simulink model "EXTENSION1"  (R2025b)
settings: Solver=FixedStepAuto  StartTime=0.0  StopTime=10.0  FixedStep=0.001  RelTol=1e-3
undefined symbols (not defined in the file): b, C, c, g, I, kb, KK, kt, l, M, m, r, Rm, sysKF
libraries: simulink x5, vrlib x3
settings Model: Creator=jitendra  LastModifiedBy=joelalfaro
settings DataIOCC: ExternalInput=getinputstruct(op_trim1)  InitialState=getstatestruct(op_trim1)  ReturnWorkspaceOutputs=off
settings DebuggingCC: UnconnectedInputMsg=warning  UnconnectedOutputMsg=warning  UnconnectedLineMsg=warning  ArithmeticOperatorsInVariantConditions=warning
settings ModelReferenceCC: EnableRefExpFcnMdlSchedulingChecks=on
settings SFSimCC: SimUseLocalCustomCode=off  CustomCodeUndefinedFunction=UseInterfaceOnly
settings RTWCC: RTWUseLocalCustomCode=off  GPUComputeCapability=3.5

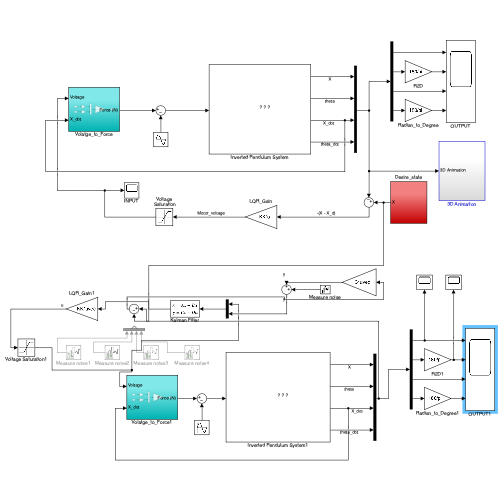
[thumbnail: Simulink's stored preview of the top-level diagram]
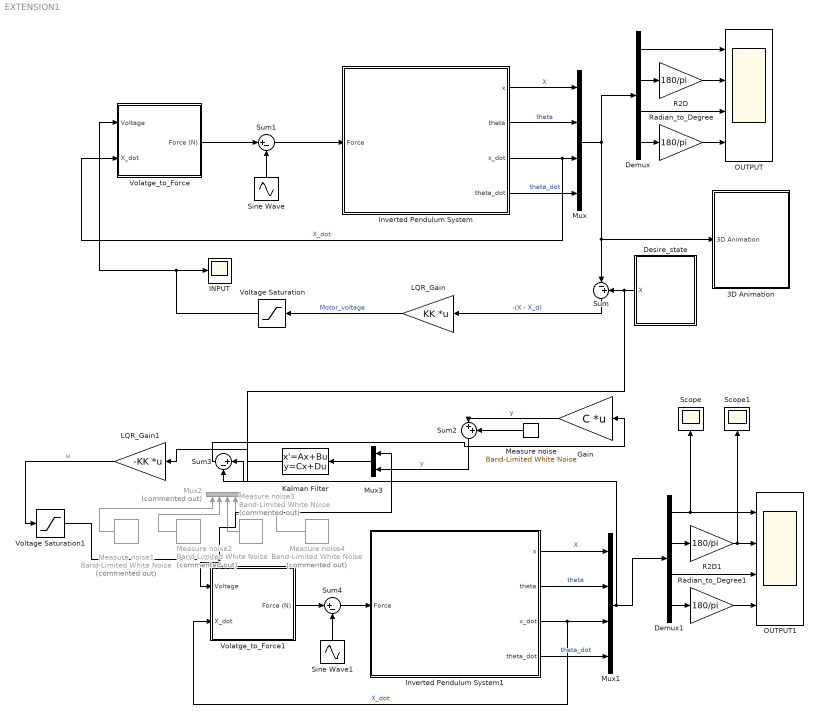
== system EXTENSION1 ==
  3D Animation : Subsystem
  Demux : Demux
  Demux1 : Demux
  Desire_state : Subsystem
  Gain : Gain  Gain=C  Multiplication=Matrix(K*u) (u vector)
  INPUT : Scope
      settings: ActiveDisplayYMinimum=-15  ActiveDisplayYMaximum=15
  Inverted Pendulum System : Subsystem
      mask Display: image('ip_model.png');
  Inverted Pendulum System1 : Subsystem
      mask Display: image('ip_model.png');
  Kalman Filter : StateSpace  A=sysKF.A  B=sysKF.B  C=sysKF.C  D=sysKF.D  InitialCondition=[0.1; 160*(pi/180)-pi; 0; 0]
  LQR_Gain : Gain  Gain=KK  Multiplication=Matrix(K*u)
  LQR_Gain1 : Gain  Gain=-KK  Multiplication=Matrix(K*u) (u vector)
  Measure noise : simulink/Sources/Band-Limited White Noise  Cov=[0]  Ts=1  seed=[23341]
  Measure noise{1..4} (4 alike) : simulink/Sources/Band-Limited White Noise  Commented=on  Cov=[0.05]  Ts=1  seed=[23341]
  Mux : Mux
  Mux1 : Mux
  Mux2 : Mux  Commented=on
  Mux3 : Mux  Inputs=2
  OUTPUT : Scope  NumInputPorts=4
      settings: ActiveDisplayString=4  ActiveDisplayYMinimum=-697.02054851210175  ActiveDisplayYMaximum=832.81658993210158  YLabel=\theta dot (deg/sec)
  OUTPUT1 : Scope  NumInputPorts=4
      settings: ActiveDisplayString=4  ActiveDisplayYMinimum=-175.01239944867373  ActiveDisplayYMaximum=256.9962748777549  YLabel=\theta dot (deg/sec)  DataLoggingVariableName=ScopeData2
  R2D : Gain  Gain=180/pi
  R2D1 : Gain  Gain=180/pi
  Radian_to_Degree : Gain  Gain=180/pi
  Radian_to_Degree1 : Gain  Gain=180/pi
  Scope : Scope
      settings: ActiveDisplayYMinimum=0.030577971463402534  ActiveDisplayYMaximum=0.77691598442287257  DataLoggingVariableName=ScopeData3
  Scope1 : Scope
      settings: ActiveDisplayYMinimum=151.06879515780136  ActiveDisplayYMaximum=200.28914360114618  DataLoggingVariableName=ScopeData4
  Sine Wave : Sin  Amplitude=0  SampleTime=0
  Sine Wave1 : Sin  Amplitude=0  SampleTime=0
  Sum : Sum  Inputs=|-+
  Sum1 : Sum  Inputs=|+-
  Sum2 : Sum  Inputs=|++
  Sum3 : Sum  Inputs=|+-
  Sum4 : Sum  Inputs=|+-
  Volatge_to_Force : Subsystem
  Volatge_to_Force1 : Subsystem
  Voltage Saturation : Saturate  UpperLimit=12  LowerLimit=-12
  Voltage Saturation1 : Saturate  UpperLimit=12  LowerLimit=-12
  wires:
  Inverted Pendulum System/3(x_dot) -> Volatge_to_Force/2(X_dot), Mux/3  "X_dot"
  Inverted Pendulum System/2(theta) -> Mux/2  "theta"
  Inverted Pendulum System/1(x) -> Mux/1  "X"
  Inverted Pendulum System/4(theta_dot) -> Mux/4  "theta_dot"
  Mux/1 -> Demux/1, Sum/1, 3D Animation/1(3D Animation)
  LQR_Gain/1 -> Voltage Saturation/1  "Motor_voltage"
  Desire_state/1(X) -> Sum/2, Sum3/2
  Sum/1 -> LQR_Gain/1  "-(X - X_d)"
  Voltage Saturation/1 -> INPUT/1, Volatge_to_Force/1(Voltage)
  Demux/2 -> R2D/1
  Demux/1 -> OUTPUT/1
  Demux/3 -> OUTPUT/3
  Demux/4 -> Radian_to_Degree/1
  R2D/1 -> OUTPUT/2
  Radian_to_Degree/1 -> OUTPUT/4
  Volatge_to_Force/1(Force (N)) -> Sum1/1
  Sum1/1 -> Inverted Pendulum System/1(Force)
  Sine Wave/1 -> Sum1/2
  Measure noise4/1 -> Mux2/4
  Radian_to_Degree1/1 -> OUTPUT1/4
  Demux1/3 -> OUTPUT1/3
  Measure noise3/1 -> Mux2/3
  Inverted Pendulum System1/1(x) -> Mux1/1  "X"
  Demux1/1 -> OUTPUT1/1, Scope/1
  Sum2/1 -> Mux3/2  "y"
  Inverted Pendulum System1/2(theta) -> Mux1/2  "theta"
  Demux1/4 -> Radian_to_Degree1/1
  Mux3/1 -> Kalman Filter/1
  Mux1/1 -> Demux1/1, Sum3/1
  Gain/1 -> Sum2/1  "y"
  Measure noise2/1 -> Mux2/2
  Inverted Pendulum System1/4(theta_dot) -> Mux1/4  "theta_dot"
  Measure noise1/1 -> Mux2/1
  R2D1/1 -> OUTPUT1/2, Scope1/1
  Demux1/2 -> R2D1/1
  Measure noise/1 -> Sum2/2
  Inverted Pendulum System1/3(x_dot) -> Volatge_to_Force1/2(X_dot), Mux1/3  "X_dot"
  Sine Wave1/1 -> Sum4/2
  Volatge_to_Force1/1(Force (N)) -> Sum4/1
  Sum4/1 -> Inverted Pendulum System1/1(Force)
  Sum3/1 -> Gain/1
  Kalman Filter/1 -> LQR_Gain1/1
  LQR_Gain1/1 -> Voltage Saturation1/1  "u"
  Voltage Saturation1/1 -> Mux3/1, Volatge_to_Force1/1(Voltage)

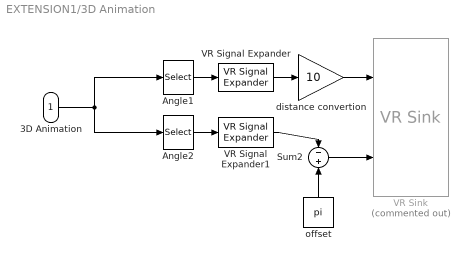
== system EXTENSION1/3D Animation ==
  3D Animation : Inport
  Angle1 : Selector  InputPortWidth=4  IndexOptions=Index vector (dialog)  Indices=[1]  OutputSizes=1
  Angle2 : Selector  InputPortWidth=4  IndexOptions=Index vector (dialog)  Indices=[2]  OutputSizes=1
  Sum2 : Sum  Inputs=-|+
  VR Signal Expander : vrlib/VR Signal Expander  outwidth=3  outidx=[1]
  VR Signal Expander1 : vrlib/VR Signal Expander  outwidth=4  outidx=[4]
  VR Sink : vrlib/VR Sink  Commented=on  InstantiateOnLoad=on  SampleTime=0.02  ViewEnable=on  RemoteChange=off  RemoteView=off  FieldsWritten=cart.translation.3.1.1.double#joint.rotation.4.1.1.double  WorldFileName=Inverted_pendulum12.wrl  AutoView=off  VideoDimensions=[]  AllowVariableSize=off  FigureProperties=[]
  distance convertion : Gain  Gain=10
  offset : Constant  Value=pi
  wires:
  VR Signal Expander/1 -> distance convertion/1
  3D Animation/1 -> Angle2/1, Angle1/1
  Angle1/1 -> VR Signal Expander/1
  Angle2/1 -> VR Signal Expander1/1
  offset/1 -> Sum2/2
  Sum2/1 -> VR Sink/2
  VR Signal Expander1/1 -> Sum2/1
  distance convertion/1 -> VR Sink/1

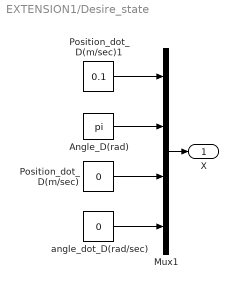
== system EXTENSION1/Desire_state ==
  Angle_D(rad) : Constant  Value=pi
  Mux1 : Mux
  Position_dot_D(m/sec) : Constant  Value=0
  Position_dot_D(m/sec)1 : Constant  Value=0.1
  angle_dot_D(rad/sec) : Constant  Value=0
  X : Outport  VectorParamsAs1DForOutWhenUnconnected=off
  wires:
  Mux1/1 -> X/1
  Position_dot_D(m/sec)/1 -> Mux1/3
  angle_dot_D(rad/sec)/1 -> Mux1/4
  Angle_D(rad)/1 -> Mux1/2
  Position_dot_D(m/sec)1/1 -> Mux1/1

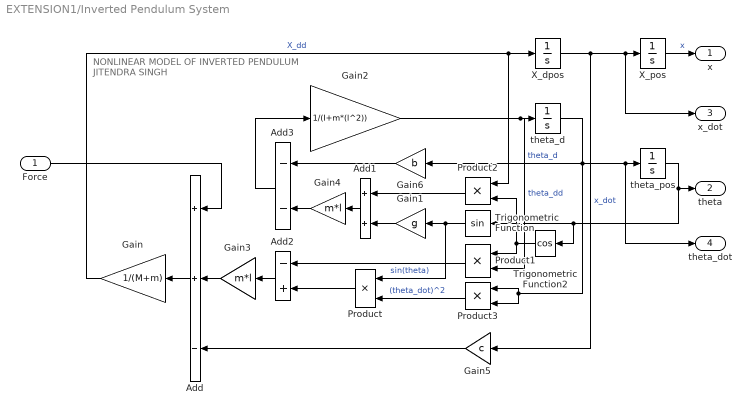
== system EXTENSION1/Inverted Pendulum System ==
  note: NONLINEAR MODEL OF
      | INVERTED PENDULUM
      | JITENDRA SINGH
  Force : Inport
  Add : Sum  Inputs=++-
  Add1 : Sum
  Add2 : Sum  Inputs=-+
  Add3 : Sum  Inputs=--
  Gain : Gain  Gain=1/(M+m)
  Gain1 : Gain  Gain=g
  Gain2 : Gain  Gain=1/(I+m*(l^2))
  Gain3 : Gain  Gain=m*l
  Gain4 : Gain  Gain=m*l
  Gain5 : Gain  Gain=c
  Gain6 : Gain  Gain=b
  Product{,1..3} (4 alike) : Product
  Trigonometric Function : Trigonometry
  Trigonometric Function2 : Trigonometry  Operator=cos
  X_dpos : Integrator
  X_pos : Integrator  InitialCondition=0.2
  theta_d : Integrator
  theta_pos : Integrator  InitialCondition=160*(pi/180)
  x : Outport  VectorParamsAs1DForOutWhenUnconnected=off
  theta : Outport  Port=2  VectorParamsAs1DForOutWhenUnconnected=off
  x_dot : Outport  Port=3  VectorParamsAs1DForOutWhenUnconnected=off
  theta_dot : Outport  Port=4  VectorParamsAs1DForOutWhenUnconnected=off
  wires:
  Gain5/1 -> Add/3
  Add2/1 -> Gain3/1
  Add3/1 -> Gain2/1
  Trigonometric Function2/1 -> Product2/2, Product1/1
  Trigonometric Function/1 -> Product/1, Gain1/1  "sin(theta)"
  Gain3/1 -> Add/2
  theta_d/1 -> Product3/2, Product3/1, Gain6/1, theta_dot/1, theta_pos/1  "theta_d"
  Product2/1 -> Add1/1
  Product/1 -> Add2/2
  Gain4/1 -> Add3/2
  Product3/1 -> Product/2  "(theta_dot)^2"
  X_pos/1 -> x/1  "x"
  Product1/1 -> Add2/1
  Gain/1 -> X_dpos/1, Product2/1  "X_dd"
  Add/1 -> Gain/1
  Gain2/1 -> Product1/2, theta_d/1  "theta_dd"
  Gain6/1 -> Add3/1
  theta_pos/1 -> Trigonometric Function2/1, Trigonometric Function/1, theta/1
  Force/1 -> Add/1
  Gain1/1 -> Add1/2
  X_dpos/1 -> x_dot/1, X_pos/1, Gain5/1  "x_dot"
  Add1/1 -> Gain4/1

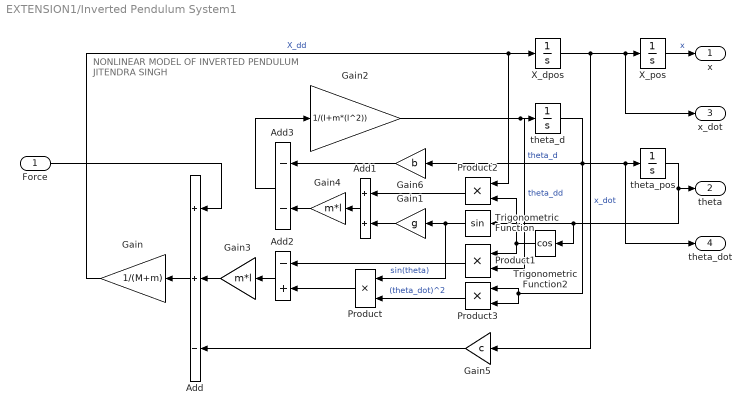
== system EXTENSION1/Inverted Pendulum System1 ==
  note: NONLINEAR MODEL OF
      | INVERTED PENDULUM
      | JITENDRA SINGH
  Force : Inport
  Add : Sum  Inputs=++-
  Add1 : Sum
  Add2 : Sum  Inputs=-+
  Add3 : Sum  Inputs=--
  Gain : Gain  Gain=1/(M+m)
  Gain1 : Gain  Gain=g
  Gain2 : Gain  Gain=1/(I+m*(l^2))
  Gain3 : Gain  Gain=m*l
  Gain4 : Gain  Gain=m*l
  Gain5 : Gain  Gain=c
  Gain6 : Gain  Gain=b
  Product{,1..3} (4 alike) : Product
  Trigonometric Function : Trigonometry
  Trigonometric Function2 : Trigonometry  Operator=cos
  X_dpos : Integrator
  X_pos : Integrator  InitialCondition=0.2
  theta_d : Integrator
  theta_pos : Integrator  InitialCondition=160*(pi/180)
  x : Outport  VectorParamsAs1DForOutWhenUnconnected=off
  theta : Outport  Port=2  VectorParamsAs1DForOutWhenUnconnected=off
  x_dot : Outport  Port=3  VectorParamsAs1DForOutWhenUnconnected=off
  theta_dot : Outport  Port=4  VectorParamsAs1DForOutWhenUnconnected=off
  wires:
  Gain5/1 -> Add/3
  Add2/1 -> Gain3/1
  Add3/1 -> Gain2/1
  Trigonometric Function2/1 -> Product2/2, Product1/1
  Trigonometric Function/1 -> Product/1, Gain1/1  "sin(theta)"
  Gain3/1 -> Add/2
  theta_d/1 -> Product3/2, Product3/1, Gain6/1, theta_dot/1, theta_pos/1  "theta_d"
  Product2/1 -> Add1/1
  Product/1 -> Add2/2
  Gain4/1 -> Add3/2
  Product3/1 -> Product/2  "(theta_dot)^2"
  X_pos/1 -> x/1  "x"
  Product1/1 -> Add2/1
  Gain/1 -> X_dpos/1, Product2/1  "X_dd"
  Add/1 -> Gain/1
  Gain2/1 -> Product1/2, theta_d/1  "theta_dd"
  Gain6/1 -> Add3/1
  theta_pos/1 -> Trigonometric Function2/1, Trigonometric Function/1, theta/1
  Force/1 -> Add/1
  Gain1/1 -> Add1/2
  X_dpos/1 -> x_dot/1, X_pos/1, Gain5/1  "x_dot"
  Add1/1 -> Gain4/1

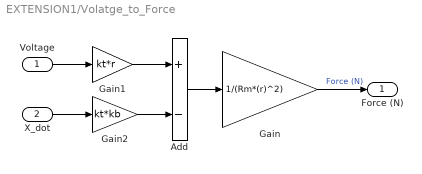
== system EXTENSION1/Volatge_to_Force ==
  Voltage : Inport
  X_dot : Inport  Port=2
  Add : Sum  Inputs=+-
  Gain : Gain  Gain=1/(Rm*(r)^2)
  Gain1 : Gain  Gain=kt*r
  Gain2 : Gain  Gain=kt*kb
  Force (N) : Outport  VectorParamsAs1DForOutWhenUnconnected=off
  wires:
  Gain1/1 -> Add/1
  Gain2/1 -> Add/2
  Voltage/1 -> Gain1/1
  Gain/1 -> Force (N)/1  "Force (N)"
  X_dot/1 -> Gain2/1
  Add/1 -> Gain/1

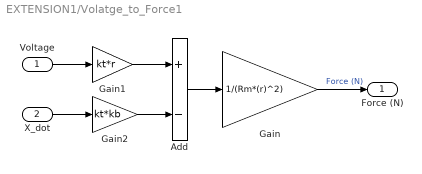
== system EXTENSION1/Volatge_to_Force1 ==
  Voltage : Inport
  X_dot : Inport  Port=2
  Add : Sum  Inputs=+-
  Gain : Gain  Gain=1/(Rm*(r)^2)
  Gain1 : Gain  Gain=kt*r
  Gain2 : Gain  Gain=kt*kb
  Force (N) : Outport  VectorParamsAs1DForOutWhenUnconnected=off
  wires:
  Gain1/1 -> Add/1
  Gain2/1 -> Add/2
  Voltage/1 -> Gain1/1
  Gain/1 -> Force (N)/1  "Force (N)"
  X_dot/1 -> Gain2/1
  Add/1 -> Gain/1
